simulink model "os4"  (R2026b)
settings: Solver=VariableStepAuto  StopTime=cel.Tsim  MaxStep=0.01
undefined symbols (not defined in the file): az, cel, el
libraries: slpidlib x2
settings Model: Creator=Alan  LastModifiedBy=Alan
settings SolverCC: ZeroCrossControl=DisableAll

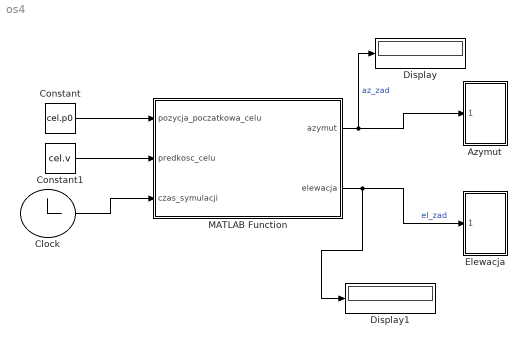
== system os4 ==
  Azymut : Subsystem
  Clock : Clock
  Constant : Constant  Value=cel.p0
  Constant1 : Constant  Value=cel.v
  Display : Display
  Display1 : Display
  Elewacja : Subsystem
  MATLAB Function : MATLAB Function  TreatAsAtomicUnit=on
  wires:
  MATLAB Function/1(azymut) -> Azymut/1(az_zadany), Display/1  "az_zad"
  MATLAB Function/2(elewacja) -> Display1/1, Elewacja/1(elewacja)  "el_zad"
  Constant1/1 -> MATLAB Function/2(predkosc_celu)
  Clock/1 -> MATLAB Function/3(czas_symulacji)
  Constant/1 -> MATLAB Function/1(pozycja_poczatkowa_celu)

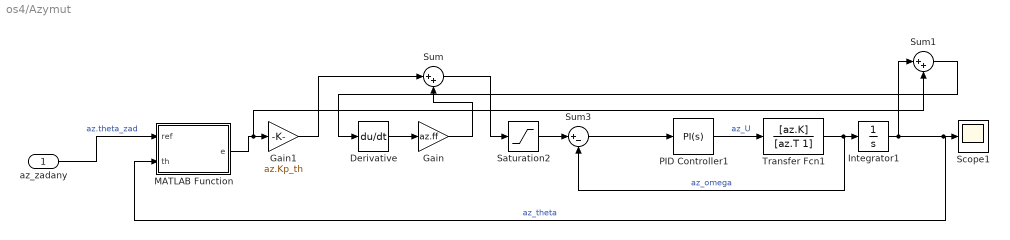
== system os4/Azymut ==
  az_zadany : Inport
  Derivative : Derivative
  Gain : Gain  Gain=az.ff
  Gain1 : Gain  Gain=az.Kp_th
  Integrator1 : Integrator  InitialCondition=az.th0
  MATLAB Function : MATLAB Function  TreatAsAtomicUnit=on
  PID Controller1 : slpidlib/PID Controller  Controller=PI  Form=Parallel  TimeDomain=Continuous-time  UseExternalTs=off  SampleTime=-1  IntegratorMethod=Forward Euler  FilterMethod=Forward Euler  ControllerParametersSource=internal  P=az.Kp_w  I=az.Ki_w  UseKiTs=off  D=0  UseExternalDerivativeSource=off  N=100  UseFilter=on  TunerSelectOption=Transfer Function Based (PID Tuner App)  InitialConditionSource=internal  InitialConditionForIntegrator=0  InitialConditionForFilter=0  DifferentiatorICPrevScaledInput=0  ExternalReset=none  TrackingMode=off  Kt=1  LimitOutput=on  SatLimitsSource=internal  UpperSaturationLimit=az.Umax  LowerSaturationLimit=-az.Umax  LinearizeAsGain=on  AntiWindupMode=clamping  Kb=1  LimitIntegrator=off  UpperIntegratorSaturationLimit=inf  LowerIntegratorSaturationLimit=-inf  POutMin=[]  POutMax=[]  IOutMin=[]  IOutMax=[]  DOutMin=[]  DOutMax=[]  NOutMin=[]  NOutMax=[]  SumOutMin=[]  SumOutMax=[]  SaturationOutMin=[]  SaturationOutMax=[]  PParamMin=[]  PParamMax=[]  IParamMin=[]  IParamMax=[]  DParamMin=[]  DParamMax=[]  NParamMin=[]  NParamMax=[]  KbParamMin=[]  KbParamMax=[]  KtParamMin=[]  KtParamMax=[]  KbOutMin=[]  KbOutMax=[]  KtOutMin=[]  KtOutMax=[]  IntegratorOutMin=[]  IntegratorOutMax=[]  FilterOutMin=[]  FilterOutMax=[]  SumI1OutMin=[]  SumI1OutMax=[]  SumI2OutMin=[]  SumI2OutMax=[]  SumI3OutMin=[]  SumI3OutMax=[]  SumI4OutMin=[]  SumI4OutMax=[]  SumDOutMin=[]  SumDOutMax=[]  DifferentiatorOutMin=[]  DifferentiatorOutMax=[]  FilterDiffOutCoefMin=[]  FilterDiffOutCoefMax=[]  ReciprocalOutMin=[]  ReciprocalOutMax=[]  SumDenOutMin=[]  SumDenOutMax=[]  SumNumOutMin=[]  SumNumOutMax=[]  DivideOutMin=[]  DivideOutMax=[]  UdiffTsProdOutMin=[]  UdiffTsProdOutMax=[]  NTsProdOutMin=[]  NTsProdOutMax=[]  UintegralTsProdOutMin=[]  UintegralTsProdOutMax=[]  UngainTsProdOutMin=[]  UngainTsProdOutMax=[]  ClampingZeroOutDataTypeStr=Inherit: Inherit via back propagation  ClampingZeroOutMin=[]  ClampingZeroOutMax=[]  FilterDenConstantOutDataTypeStr=Inherit: Inherit via back propagation  FilterDenConstantOutMin=[]  FilterDenConstantOutMax=[]  PCopyOutDataTypeStr=Inherit: Inherit via back propagation  PCopyOutMin=[]  PCopyOutMax=[]  NCopyOutDataTypeStr=Inherit: Inherit via back propagation  NCopyOutMin=[]  NCopyOutMax=[]  IntegratorContinuousStateAttributes=''  IntegratorStateMustResolveToSignalObject=off  IntegratorRTWStateStorageClass=Auto  FilterContinuousStateAttributes=''  FilterStateMustResolveToSignalObject=off  FilterRTWStateStorageClass=Auto  ParallelPVariant=InternalParameters  IdealPVariant=Disabled  IVariant=InternalParameters  DVariant=Disabled  IntegratorVariant=Continuous  SatVariant=Enabled  AWVariant=ContClampingParallel  PCopyVariant=Disabled  TRVariant=Disabled  FdbkBlocksVariant=Forward  IdealPFdbkVariant=Disabled  SatFdbkVariant=Disabled  DerivativeFilterVariant=Disabled  NVariant=Disabled  NCopyVariant=Disabled_SignalSpec  FilterICVariant=Disabled  IntegratorICVariant=InternalICs  ExternalResetVariant=Disabled  TRSumVariant=Passthrough  SumFdbkVariant=Disabled  SumVariant=Sum_PI  TsampFilterVariant=InternalTs  TsampNgainVariant=Passthrough  TsampIntegralVariant=Disabled_SignalSpec  ExternalSaturationOutDataTypeStr=Inherit: Same as second input  DerivativeSourceVariant=Disabled  PreIntVariant=InternalPreInt
  Saturation2 : Saturate  UpperLimit=az.wmax  LowerLimit=-az.wmax
  Scope1 : Scope
      settings: ActiveDisplayYMinimum=-7.1720754936863269  ActiveDisplayYMaximum=18.353555756313906
  Sum : Sum  Inputs=|++
  Sum1 : Sum  Inputs=|++
  Sum3 : Sum  Inputs=|+-
  Transfer Fcn1 : TransferFcn  Numerator=[az.K]  Denominator=[az.T 1]
  wires:
  Saturation2/1 -> Sum3/1
  MATLAB Function/1(e) -> Sum1/2, Gain1/1
  Transfer Fcn1/1 -> Sum3/2, Integrator1/1  "az_omega"
  Sum3/1 -> PID Controller1/1
  PID Controller1/1 -> Transfer Fcn1/1  "az_U"
  Integrator1/1 -> Sum1/1, MATLAB Function/2(th), Scope1/1  "az_theta"
  az_zadany/1 -> MATLAB Function/1(ref)  "az.theta_zad"
  Derivative/1 -> Gain/1
  Gain1/1 -> Sum/1
  Gain/1 -> Sum/2
  Sum/1 -> Saturation2/1
  Sum1/1 -> Derivative/1

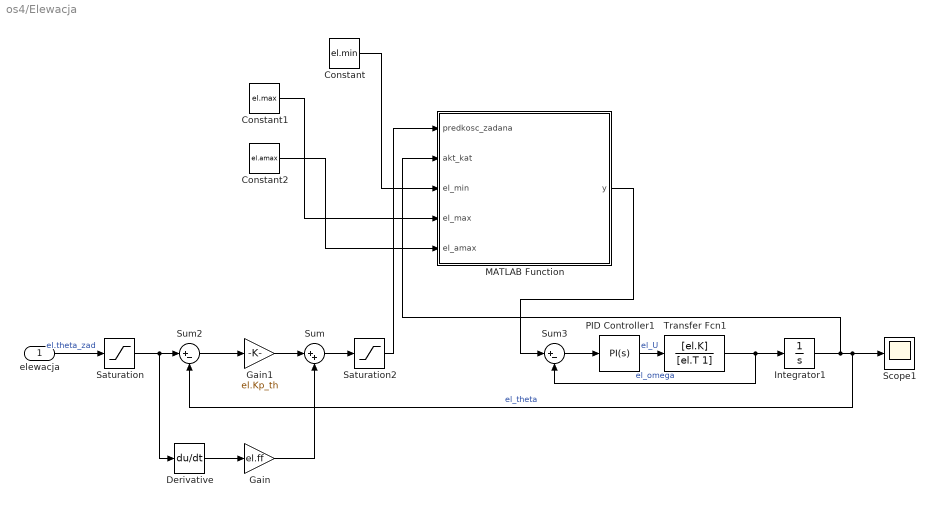
== system os4/Elewacja ==
  elewacja : Inport
  Constant : Constant  Value=el.min
  Constant1 : Constant  Value=el.max
  Constant2 : Constant  Value=el.amax
  Derivative : Derivative
  Gain : Gain  Gain=el.ff
  Gain1 : Gain  Gain=el.Kp_th
  Integrator1 : Integrator  InitialCondition=el.th0  LimitOutput=on  UpperSaturationLimit=el.stop_max  LowerSaturationLimit=el.stop_min
  MATLAB Function : MATLAB Function  TreatAsAtomicUnit=on
  PID Controller1 : slpidlib/PID Controller  Controller=PI  Form=Parallel  TimeDomain=Continuous-time  UseExternalTs=off  SampleTime=-1  IntegratorMethod=Forward Euler  FilterMethod=Forward Euler  ControllerParametersSource=internal  P=el.Kp_w  I=el.Ki_w  UseKiTs=off  D=0  UseExternalDerivativeSource=off  N=100  UseFilter=on  TunerSelectOption=Transfer Function Based (PID Tuner App)  InitialConditionSource=internal  InitialConditionForIntegrator=0  InitialConditionForFilter=0  DifferentiatorICPrevScaledInput=0  ExternalReset=none  TrackingMode=off  Kt=1  LimitOutput=on  SatLimitsSource=internal  UpperSaturationLimit=el.Umax  LowerSaturationLimit=-el.Umax  LinearizeAsGain=on  AntiWindupMode=clamping  Kb=1  LimitIntegrator=off  UpperIntegratorSaturationLimit=inf  LowerIntegratorSaturationLimit=-inf  POutMin=[]  POutMax=[]  IOutMin=[]  IOutMax=[]  DOutMin=[]  DOutMax=[]  NOutMin=[]  NOutMax=[]  SumOutMin=[]  SumOutMax=[]  SaturationOutMin=[]  SaturationOutMax=[]  PParamMin=[]  PParamMax=[]  IParamMin=[]  IParamMax=[]  DParamMin=[]  DParamMax=[]  NParamMin=[]  NParamMax=[]  KbParamMin=[]  KbParamMax=[]  KtParamMin=[]  KtParamMax=[]  KbOutMin=[]  KbOutMax=[]  KtOutMin=[]  KtOutMax=[]  IntegratorOutMin=[]  IntegratorOutMax=[]  FilterOutMin=[]  FilterOutMax=[]  SumI1OutMin=[]  SumI1OutMax=[]  SumI2OutMin=[]  SumI2OutMax=[]  SumI3OutMin=[]  SumI3OutMax=[]  SumI4OutMin=[]  SumI4OutMax=[]  SumDOutMin=[]  SumDOutMax=[]  DifferentiatorOutMin=[]  DifferentiatorOutMax=[]  FilterDiffOutCoefMin=[]  FilterDiffOutCoefMax=[]  ReciprocalOutMin=[]  ReciprocalOutMax=[]  SumDenOutMin=[]  SumDenOutMax=[]  SumNumOutMin=[]  SumNumOutMax=[]  DivideOutMin=[]  DivideOutMax=[]  UdiffTsProdOutMin=[]  UdiffTsProdOutMax=[]  NTsProdOutMin=[]  NTsProdOutMax=[]  UintegralTsProdOutMin=[]  UintegralTsProdOutMax=[]  UngainTsProdOutMin=[]  UngainTsProdOutMax=[]  ClampingZeroOutDataTypeStr=Inherit: Inherit via back propagation  ClampingZeroOutMin=[]  ClampingZeroOutMax=[]  FilterDenConstantOutDataTypeStr=Inherit: Inherit via back propagation  FilterDenConstantOutMin=[]  FilterDenConstantOutMax=[]  PCopyOutDataTypeStr=Inherit: Inherit via back propagation  PCopyOutMin=[]  PCopyOutMax=[]  NCopyOutDataTypeStr=Inherit: Inherit via back propagation  NCopyOutMin=[]  NCopyOutMax=[]  IntegratorContinuousStateAttributes=''  IntegratorStateMustResolveToSignalObject=off  IntegratorRTWStateStorageClass=Auto  FilterContinuousStateAttributes=''  FilterStateMustResolveToSignalObject=off  FilterRTWStateStorageClass=Auto  ParallelPVariant=InternalParameters  IdealPVariant=Disabled  IVariant=InternalParameters  DVariant=Disabled  IntegratorVariant=Continuous  SatVariant=Enabled  AWVariant=ContClampingParallel  PCopyVariant=Disabled  TRVariant=Disabled  FdbkBlocksVariant=Forward  IdealPFdbkVariant=Disabled  SatFdbkVariant=Disabled  DerivativeFilterVariant=Disabled  NVariant=Disabled  NCopyVariant=Disabled_SignalSpec  FilterICVariant=Disabled  IntegratorICVariant=InternalICs  ExternalResetVariant=Disabled  TRSumVariant=Passthrough  SumFdbkVariant=Disabled  SumVariant=Sum_PI  TsampFilterVariant=InternalTs  TsampNgainVariant=Passthrough  TsampIntegralVariant=Disabled_SignalSpec  ExternalSaturationOutDataTypeStr=Inherit: Same as second input  DerivativeSourceVariant=Disabled  PreIntVariant=InternalPreInt
  Saturation : Saturate  UpperLimit=el.max  LowerLimit=el.min
  Saturation2 : Saturate  UpperLimit=el.wmax  LowerLimit=-el.wmax
  Scope1 : Scope
      settings: ActiveDisplayYMinimum=-1.2189298085220446  ActiveDisplayYMaximum=4.1925574296303969
  Sum : Sum  Inputs=|++
  Sum2 : Sum  Inputs=|+-
  Sum3 : Sum  Inputs=|+-
  Transfer Fcn1 : TransferFcn  Numerator=[el.K]  Denominator=[el.T 1]
  wires:
  Transfer Fcn1/1 -> Sum3/2, Integrator1/1  "el_omega"
  Sum3/1 -> PID Controller1/1
  Integrator1/1 -> MATLAB Function/2(akt_kat), Sum2/2, Scope1/1  "el_theta"
  PID Controller1/1 -> Transfer Fcn1/1  "el_U"
  elewacja/1 -> Saturation/1  "el.theta_zad"
  Saturation/1 -> Derivative/1, Sum2/1
  Saturation2/1 -> MATLAB Function/1(predkosc_zadana)
  MATLAB Function/1(y) -> Sum3/1
  Constant/1 -> MATLAB Function/3(el_min)
  Constant1/1 -> MATLAB Function/4(el_max)
  Constant2/1 -> MATLAB Function/5(el_amax)
  Sum/1 -> Saturation2/1
  Sum2/1 -> Gain1/1
  Gain1/1 -> Sum/1
  Derivative/1 -> Gain/1
  Gain/1 -> Sum/2

== matlab function os4/Elewacja/MATLAB Function ==
  data: predkosc_zadana input; y output; akt_kat input; el_min input; el_max input; el_amax input
function y = fcn(predkosc_zadana, akt_kat, el_min, el_max, el_amax)

    s_gora = el_max - akt_kat;
    s_dol = akt_kat - el_min;
    w_gora = sqrt(2*el_amax*max(s_gora,0));
    w_dol = sqrt(2*el_amax*max(s_dol,0));

    w_ogr = min(predkosc_zadana, w_gora);   % nie szybciej niz w_gora w gore
    y = max(w_ogr, -w_dol);             % nie szybciej niz w_dol w dol

== matlab function os4/Azymut/MATLAB Function ==
  data: ref input; e output; th input
function e = uchyb_kolowy(ref, th)
% Uchyb azymutu zawiniety do przedzialu (-pi, pi]:
% lufa zawsze obraca sie najkrotsza droga.
e = mod(ref - th + pi, 2*pi) - pi;
end

== matlab function os4/MATLAB Function ==
  data: pozycja_poczatkowa_celu input; azymut output; predkosc_celu input; czas_symulacji input; elewacja output
function [azymut,elewacja] = fcn(pozycja_poczatkowa_celu, predkosc_celu, czas_symulacji)



p = pozycja_poczatkowa_celu+predkosc_celu*czas_symulacji;
c = sqrt(power(p(1),2)+power(p(2),2));
azymut = mod(atan2(p(1), p(2)), 2*pi);
elewacja = atan2(p(3),c);
